simulink model "AFC_FFNN_trainbfg_15_15_15_15_ctr_Nor_July_15"  (R2023a)
settings: Solver=VariableStepAuto  StartTime=0.0  StopTime=10.0  RelTol=1e-3
libraries: neural x66
(part 2 of 3)

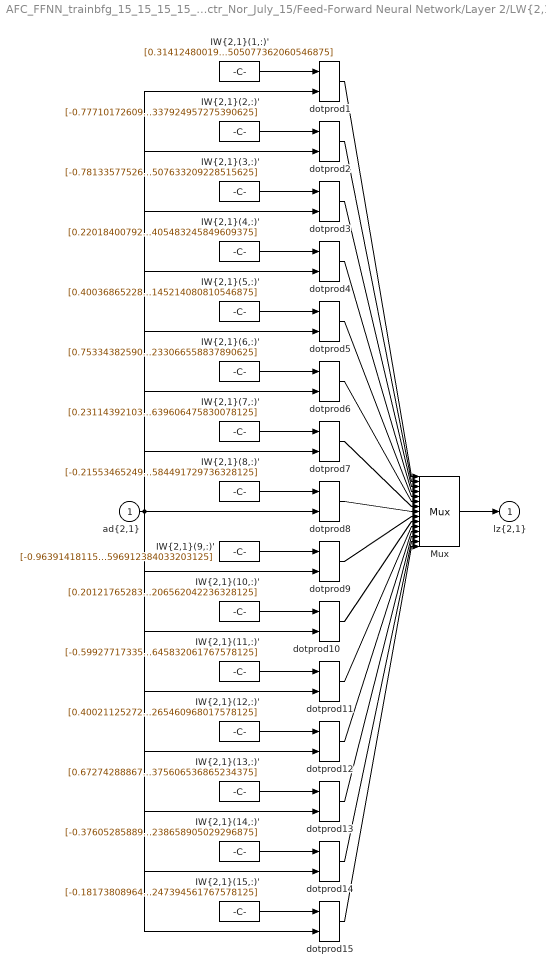
== system AFC_FFNN_trainbfg_15_15_15_15_ctr_Nor_July_15/Feed-Forward Neural Network/Layer 2/LW{2,1} ==
  "ad{2,1}" : Inport  PortDimensions=15
      mask Display: e = 0.06;c1 = [120 230 180]/255;c2 = ([120 230 180]+0)/(256+128);c3 = ([120 230 180]+128)/(256+128);patch([0 1 1 0],[0 0 1 1],c1);patch([0 1 1 1-e 1-e 0+e],[0 0 1 1-e 0+e 0+e],c2);patch([0 0 1 1-e 0+e 0+e],[0 1 1 1-e 1-e 0+e],c3);plot([0 1 1 0 0],[0 0 1 1 0]);
  "IW{2,1}(1,:)'" : Constant  Value=[0.314124800191435848972787425736896693706512451171875;0.761219194780894614638100392767228186130523681640625;-0.171753869070582876332764499238692224025726318359375;0.1327757115322516501265681654331274330615997314453125;0.2459442725020564157745184274972416460514068603515625;0.7167434795542131364953775118920020759105682373046875;-0.4743644560107054264364023765665479004383087158203125;0.9964541018726646992575979311368428170680999755859375;-0.3007178641450372058585571721778251230716705322265625;-0.5061911842499977609577399562112987041473388671875;-0.6212526524824333318264280023868195712566375732421875;-0.32664100949461083445157782989554107189178466796875;-0.164745119790139948889873267035000026226043701171875;-0.37571726232811375467690595542080700397491455078125;-0.9219376696445731322882011227193288505077362060546875]
      mask Display: e = 0.06;c1 = [120 150 230]/255;c2 = ([120 150 230]+0)/383;c3 = ([120 150 230]+128)/383;patch([0 1 1 0],[0 0 1 1],c1);patch([0 1 1 1-e 1-e 0+e],[0 0 1 1-e 0+e 0+e],c2);patch([0 0 1 1-e 0+e 0+e],[0 1 1 1-e 1-e 0+e],c3);plot([0 1 1 0 0],[0 0 1 1 0]);disp('weights');
  "IW{2,1}(10,:)'" : Constant  Value=[0.201217652832927473838253717985935509204864501953125;0.7240782555431468647810788752394728362560272216796875;0.8421596785908558313593630373361520469188690185546875;-1.1825149875412674926877798498026095330715179443359375;-0.31519109748938467507883842699811793863773345947265625;-0.795521501318470658503656522952951490879058837890625;0.0713141598183908431707322961301542818546295166015625;-0.0767485023139631294952778262086212635040283203125;-0.1010553699979890307503183066728524863719940185546875;-0.9567843225283756414256686184671707451343536376953125;-0.7217264190297532078233189167804084718227386474609375;0.50100226468314923433666763230576179921627044677734375;0.87766383555333093990924453464685939252376556396484375;0.29681483600678404410899702270398847758769989013671875;0.2310269064815640149834763406033744104206562042236328125]
      mask Display: e = 0.06;c1 = [120 150 230]/255;c2 = ([120 150 230]+0)/383;c3 = ([120 150 230]+128)/383;patch([0 1 1 0],[0 0 1 1],c1);patch([0 1 1 1-e 1-e 0+e],[0 0 1 1-e 0+e 0+e],c2);patch([0 0 1 1-e 0+e 0+e],[0 1 1 1-e 1-e 0+e],c3);plot([0 1 1 0 0],[0 0 1 1 0]);disp('weights');
  "IW{2,1}(11,:)'" : Constant  Value=[-0.5992771733562098912528881555772386491298675537109375;0.1078487493560353893684577997191809117794036865234375;-0.8945967236389289478637465435895137488842010498046875;-0.0500773407099595058156182858510874211788177490234375;0.8870816241124896972536362227401696145534515380859375;0.74014207030404488563135600998066365718841552734375;-0.6866720030229107596397852830705232918262481689453125;0.2726234239649603097177532617934048175811767578125;0.2078428359638626599092958713299594819545745849609375;0.1188907111891503998180041890009306371212005615234375;-0.469008120701347674952330635278485715389251708984375;-0.37068355488443938128284571575932204723358154296875;-0.123525625729133281538452138192951679229736328125;-0.58507783620791808942840361851267516613006591796875;-0.222821272390497870929948476259596645832061767578125]
      mask Display: e = 0.06;c1 = [120 150 230]/255;c2 = ([120 150 230]+0)/383;c3 = ([120 150 230]+128)/383;patch([0 1 1 0],[0 0 1 1],c1);patch([0 1 1 1-e 1-e 0+e],[0 0 1 1-e 0+e 0+e],c2);patch([0 0 1 1-e 0+e 0+e],[0 1 1 1-e 1-e 0+e],c3);plot([0 1 1 0 0],[0 0 1 1 0]);disp('weights');
  "IW{2,1}(12,:)'" : Constant  Value=[0.4002112527225698546118337617372162640094757080078125;0.6440325108893374395080400063307024538516998291015625;0.2318822635474317994663806530297733843326568603515625;-1.2667374338708261571895263841724954545497894287109375;-0.5533384432674870456736471169278956949710845947265625;-0.26613616681114093953652854906977154314517974853515625;0.3727253587085710417881045941612683236598968505859375;0.48813811599891376857840441516600549221038818359375;0.6001589125458657303369136570836417376995086669921875;-0.0802101438462316795874329500293242745101451873779296875;0.65367435221139091883202354438253678381443023681640625;-1.0458216791451082627872892771847546100616455078125;-1.3193113394946169858457096779602579772472381591796875;-0.330369571278571971806314877539989538490772247314453125;0.997369857636166035064206880633719265460968017578125]
      mask Display: e = 0.06;c1 = [120 150 230]/255;c2 = ([120 150 230]+0)/383;c3 = ([120 150 230]+128)/383;patch([0 1 1 0],[0 0 1 1],c1);patch([0 1 1 1-e 1-e 0+e],[0 0 1 1-e 0+e 0+e],c2);patch([0 0 1 1-e 0+e 0+e],[0 1 1 1-e 1-e 0+e],c3);plot([0 1 1 0 0],[0 0 1 1 0]);disp('weights');
  "IW{2,1}(13,:)'" : Constant  Value=[0.67274288867184051099457064992748200893402099609375;0.189393636354295846757622712175361812114715576171875;-0.510549226010743151249471338815055787563323974609375;1.104023685506638319253625013516284525394439697265625;0.8308657357789719366536473899031989276409149169921875;0.367241219801807627920453569458913989365100860595703125;0.8655885705956922748782744747586548328399658203125;-0.0858121130468900705778878545970655977725982666015625;-0.8378375318602981902671444913721643388271331787109375;-0.88685905025613409602414094479172490537166595458984375;0.275859743807580104490995154264965094625949859619140625;0.2062969216335570621367878629826009273529052734375;1.1086902941997625049452835810370743274688720703125;0.442383535765201452161221595815732143819332122802734375;0.95884080775527402717983704860671423375606536865234375]
      mask Display: e = 0.06;c1 = [120 150 230]/255;c2 = ([120 150 230]+0)/383;c3 = ([120 150 230]+128)/383;patch([0 1 1 0],[0 0 1 1],c1);patch([0 1 1 1-e 1-e 0+e],[0 0 1 1-e 0+e 0+e],c2);patch([0 0 1 1-e 0+e 0+e],[0 1 1 1-e 1-e 0+e],c3);plot([0 1 1 0 0],[0 0 1 1 0]);disp('weights');
  "IW{2,1}(14,:)'" : Constant  Value=[-0.3760528588983949038748733073589392006397247314453125;-0.3766582837641696546171488080290146172046661376953125;0.9248846167847240007375830828095786273479461669921875;-0.8676145111114246244454761836095713078975677490234375;0.157385168877649583851763281927560456097126007080078125;-0.4984382819952763998827549585257656872272491455078125;-0.07612045846803727755514046293683350086212158203125;0.1706855767497774678531641256995499134063720703125;0.6769974800018092597753138761618174612522125244140625;0.5403602376259268869063134843599982559680938720703125;-2.3605068409971039500305778346955776214599609375;-0.16106471547288514489792987660621292889118194580078125;-0.369042109842184939960674228132120333611965179443359375;-0.95704290874445641090773051473661325871944427490234375;0.843577088247318140901143124210648238658905029296875]
      mask Display: e = 0.06;c1 = [120 150 230]/255;c2 = ([120 150 230]+0)/383;c3 = ([120 150 230]+128)/383;patch([0 1 1 0],[0 0 1 1],c1);patch([0 1 1 1-e 1-e 0+e],[0 0 1 1-e 0+e 0+e],c2);patch([0 0 1 1-e 0+e 0+e],[0 1 1 1-e 1-e 0+e],c3);plot([0 1 1 0 0],[0 0 1 1 0]);disp('weights');
  "IW{2,1}(15,:)'" : Constant  Value=[-0.1817380896437239545804231966030783951282501220703125;-0.819076525749918626928547382703982293605804443359375;-0.703422130964734382274627932929433882236480712890625;-0.94939269002778214900928333008778281509876251220703125;-0.896269677871021741566437412984669208526611328125;-0.3356003910290790148707174012088216841220855712890625;-0.2214840900786894106744284727028571069240570068359375;-0.4191414392946388733918183788773603737354278564453125;-0.2687179919619584467227468849159777164459228515625;0.98276969821900905799338943324983119964599609375;-0.0363505221006390488724946408183313906192779541015625;-0.55328677456039410120780530633055604994297027587890625;0.89155338038898801489295919964206404983997344970703125;-0.11752903231500504144246832538556191138923168182373046875;-0.79833567739331734447461030867998488247394561767578125]
      mask Display: e = 0.06;c1 = [120 150 230]/255;c2 = ([120 150 230]+0)/383;c3 = ([120 150 230]+128)/383;patch([0 1 1 0],[0 0 1 1],c1);patch([0 1 1 1-e 1-e 0+e],[0 0 1 1-e 0+e 0+e],c2);patch([0 0 1 1-e 0+e 0+e],[0 1 1 1-e 1-e 0+e],c3);plot([0 1 1 0 0],[0 0 1 1 0]);disp('weights');
  "IW{2,1}(2,:)'" : Constant  Value=[-0.7771017260971981865935731548233889043331146240234375;-0.989689411673975616423604151350446045398712158203125;0.85939642766992552225246981834061443805694580078125;-0.61030381879570694270142894310993142426013946533203125;0.30497898667072576017744722776114940643310546875;0.092222522227818071183236270371708087623119354248046875;-0.005466530920209766719608523999340832233428955078125;0.8236928328595840564929631000268273055553436279296875;0.0456944657569839929323052274412475526332855224609375;0.8261448944639935287881371550611220300197601318359375;0.429014213658457210787133817575522698462009429931640625;-0.32131717688586680647944149313843809068202972412109375;-0.52240941017245867694640537592931650578975677490234375;0.29152713968148391554535692193894647061824798583984375;0.494308555574343666538794650477939285337924957275390625]
      mask Display: e = 0.06;c1 = [120 150 230]/255;c2 = ([120 150 230]+0)/383;c3 = ([120 150 230]+128)/383;patch([0 1 1 0],[0 0 1 1],c1);patch([0 1 1 1-e 1-e 0+e],[0 0 1 1-e 0+e 0+e],c2);patch([0 0 1 1-e 0+e 0+e],[0 1 1 1-e 1-e 0+e],c3);plot([0 1 1 0 0],[0 0 1 1 0]);disp('weights');
  "IW{2,1}(3,:)'" : Constant  Value=[-0.7813357752653991017410817221389152109622955322265625;0.2884373573340142105081440604408271610736846923828125;-0.1790504980917517752203593772719614207744598388671875;-0.62459444844897393789295847454923205077648162841796875;0.9792166972620892639866951867588795721530914306640625;-0.05772109104215349117961153524447581730782985687255859375;-0.0859133263877100983307855130988173186779022216796875;-0.903421362694661223002867700415663421154022216796875;-0.3519069100123857207762512189219705760478973388671875;0.68567142254128310430161263866466470062732696533203125;0.427114206938296436799618049917626194655895233154296875;-0.1887415273689747596819188402150757610797882080078125;0.08611314277500585478986039333904045633971691131591796875;0.9918392466822412156801647142856381833553314208984375;-0.8345158850484593049401382813812233507633209228515625]
      mask Display: e = 0.06;c1 = [120 150 230]/255;c2 = ([120 150 230]+0)/383;c3 = ([120 150 230]+128)/383;patch([0 1 1 0],[0 0 1 1],c1);patch([0 1 1 1-e 1-e 0+e],[0 0 1 1-e 0+e 0+e],c2);patch([0 0 1 1-e 0+e 0+e],[0 1 1 1-e 1-e 0+e],c3);plot([0 1 1 0 0],[0 0 1 1 0]);disp('weights');
  "IW{2,1}(4,:)'" : Constant  Value=[0.22018400792110437436122083454392850399017333984375;0.6991144072415418353472205126308836042881011962890625;0.3099402980647762984034443434211425483226776123046875;0.061498952364746749255086655239210813306272029876708984375;0.439963017584670768034271759461262263357639312744140625;0.53700087765160320341095712137757800519466400146484375;-0.9259617635520160927597999034333042800426483154296875;0.6153389276731864310221453706617467105388641357421875;-0.4045481598141231760479286094778217375278472900390625;0.70229649611518774054985669863526709377765655517578125;-1.0632415478873624703481937103788368403911590576171875;1.037732974579840483642101389705203473567962646484375;-0.56732075540575477301530327167711220681667327880859375;0.03649661653649223513884436442822334356606006622314453125;0.6470024656570847465530960107571445405483245849609375]
      mask Display: e = 0.06;c1 = [120 150 230]/255;c2 = ([120 150 230]+0)/383;c3 = ([120 150 230]+128)/383;patch([0 1 1 0],[0 0 1 1],c1);patch([0 1 1 1-e 1-e 0+e],[0 0 1 1-e 0+e 0+e],c2);patch([0 0 1 1-e 0+e 0+e],[0 1 1 1-e 1-e 0+e],c3);plot([0 1 1 0 0],[0 0 1 1 0]);disp('weights');
  "IW{2,1}(5,:)'" : Constant  Value=[0.4003686522850926632344226163695566356182098388671875;0.7154922757569484037531992726144380867481231689453125;-0.55451457198497333678233189857564866542816162109375;-0.701016426748160892401529054041020572185516357421875;0.2719693029116949656298629633965902030467987060546875;0.3452701580345747256473032393842004239559173583984375;-0.9904793588654232650014819228090345859527587890625;0.421753225196830339172038293327204883098602294921875;-0.6134849306530993917618843624950386583805084228515625;0.6205332793438713689937458184431307017803192138671875;-0.2900360464848421582217952163773588836193084716796875;-0.8601594396824143728963463217951357364654541015625;-0.7387104842103118240714820785797201097011566162109375;-0.64540323855050463208726796437986195087432861328125;-0.2133330335187888504577813364448957145214080810546875]
      mask Display: e = 0.06;c1 = [120 150 230]/255;c2 = ([120 150 230]+0)/383;c3 = ([120 150 230]+128)/383;patch([0 1 1 0],[0 0 1 1],c1);patch([0 1 1 1-e 1-e 0+e],[0 0 1 1-e 0+e 0+e],c2);patch([0 0 1 1-e 0+e 0+e],[0 1 1 1-e 1-e 0+e],c3);plot([0 1 1 0 0],[0 0 1 1 0]);disp('weights');
  "IW{2,1}(6,:)'" : Constant  Value=[0.7533438259077460674717485744622536003589630126953125;-0.1622850437559437697387920707114972174167633056640625;-0.2221844078714447778821750034694559872150421142578125;0.54429151285718668784596729892655275762081146240234375;1.00787934291988801049910762230865657329559326171875;0.3163128591791328769744495730265043675899505615234375;0.2893143771285426879558144719339907169342041015625;0.9802256885177147438525935285724699497222900390625;-0.3613982857657287439678839291445910930633544921875;-0.90323576071038391699374869858729653060436248779296875;1.52266978362477178876588368439115583896636962890625;0.414545013788929994635878983899601735174655914306640625;-0.25805726547611007593019394334987737238407135009765625;0.79414819953845261490954499095096252858638763427734375;0.465672824324343537227832712233066558837890625]
      mask Display: e = 0.06;c1 = [120 150 230]/255;c2 = ([120 150 230]+0)/383;c3 = ([120 150 230]+128)/383;patch([0 1 1 0],[0 0 1 1],c1);patch([0 1 1 1-e 1-e 0+e],[0 0 1 1-e 0+e 0+e],c2);patch([0 0 1 1-e 0+e 0+e],[0 1 1 1-e 1-e 0+e],c3);plot([0 1 1 0 0],[0 0 1 1 0]);disp('weights');
  "IW{2,1}(7,:)'" : Constant  Value=[0.23114392103916969745114329271018505096435546875;0.9635763073263967637416271827532909810543060302734375;-0.1671208207308916282585187218501232564449310302734375;0.06329895739177394953234312424683594144880771636962890625;-0.378452929134685034373575263089151121675968170166015625;0.11958422424242327875010261095667374320328235626220703125;-0.607419333399665362094310694374144077301025390625;0.0111096917961808205888019074336625635623931884765625;-0.8105754243397400582438194760470651090145111083984375;0.318929817605345056197307940237806178629398345947265625;-0.7900852178016195548337918808101676404476165771484375;-0.21373528018232745839810604593367315828800201416015625;-0.5969408965863836069587478050380013883113861083984375;-0.90852813610887828144058175894315354526042938232421875;-0.287242937260107134012088181407307274639606475830078125]
      mask Display: e = 0.06;c1 = [120 150 230]/255;c2 = ([120 150 230]+0)/383;c3 = ([120 150 230]+128)/383;patch([0 1 1 0],[0 0 1 1],c1);patch([0 1 1 1-e 1-e 0+e],[0 0 1 1-e 0+e 0+e],c2);patch([0 0 1 1-e 0+e 0+e],[0 1 1 1-e 1-e 0+e],c3);plot([0 1 1 0 0],[0 0 1 1 0]);disp('weights');
  "IW{2,1}(8,:)'" : Constant  Value=[-0.2155346524932839624710823045461438596248626708984375;0.890530830596826472600469060125760734081268310546875;-0.9467920414380841531709620539913885295391082763671875;-0.434011281189908115774045427315286360681056976318359375;0.26579035938519302018079315530485473573207855224609375;0.2172980620921392269639937921965611167252063751220703125;0.292716250101574093633871598285622894763946533203125;0.1305612562825471112404329687706194818019866943359375;-0.871055828832263845384886735701002180576324462890625;-0.17721316472024450927591487925383262336254119873046875;-0.71934773715706235019951009235228411853313446044921875;0.25931984951627884417035829756059683859348297119140625;0.21468822963550027171919509783037938177585601806640625;0.16340570924226149873703661796753294765949249267578125;-0.81406715037500021470151523317326791584491729736328125]
      mask Display: e = 0.06;c1 = [120 150 230]/255;c2 = ([120 150 230]+0)/383;c3 = ([120 150 230]+128)/383;patch([0 1 1 0],[0 0 1 1],c1);patch([0 1 1 1-e 1-e 0+e],[0 0 1 1-e 0+e 0+e],c2);patch([0 0 1 1-e 0+e 0+e],[0 1 1 1-e 1-e 0+e],c3);plot([0 1 1 0 0],[0 0 1 1 0]);disp('weights');
  "IW{2,1}(9,:)'" : Constant  Value=[-0.96391418115658300536097158328630030155181884765625;0.510168063185229225808825503918342292308807373046875;0.312107034951037309866705982130952179431915283203125;0.33415533498262950384827263405895791947841644287109375;0.159088574682244077163062456747866235673427581787109375;0.303936777339137431663829147510114125907421112060546875;-0.06134999454679768149389929021708667278289794921875;-0.769981108969951311138402161304838955402374267578125;-0.5287401885702369686015344996121712028980255126953125;-0.0309998749507064234876008157471005688421428203582763671875;0.18321056239390876019257348161772824823856353759765625;0.0783758268001817637316008813286316581070423126220703125;0.1645435635146068609202529842150397598743438720703125;-1.1439631090601272145335087770945392549037933349609375;0.74931802165753680355919641442596912384033203125]
      mask Display: e = 0.06;c1 = [120 150 230]/255;c2 = ([120 150 230]+0)/383;c3 = ([120 150 230]+128)/383;patch([0 1 1 0],[0 0 1 1],c1);patch([0 1 1 1-e 1-e 0+e],[0 0 1 1-e 0+e 0+e],c2);patch([0 0 1 1-e 0+e 0+e],[0 1 1 1-e 1-e 0+e],c3);plot([0 1 1 0 0],[0 0 1 1 0]);disp('weights');
  Mux : Mux  Inputs=15
      mask Display: e = 0.06;c1 = [120 150 230]/255;c2 = ([120 150 230]+0)/383;c3 = ([120 150 230]+128)/383;patch([0 1 1 0],[0 0 1 1],c1);patch([0 1 1 1-e 1-e 0+e],[0 0 1 1-e 0+e 0+e],c2);patch([0 0 1 1-e 0+e 0+e],[0 1 1 1-e 1-e 0+e],c3);plot([0 1 1 0 0],[0 0 1 1 0]);disp('Mux');
  dotprod{1..15} (15 alike) : neural/Weight Functions/dotprod
  "lz{2,1}" : Outport
      mask Display: e = 0.06;c1 = [120 230 180]/255;c2 = ([120 230 180]+0)/(256+128);c3 = ([120 230 180]+128)/(256+128);patch([0 1 1 0],[0 0 1 1],c1);patch([0 1 1 1-e 1-e 0+e],[0 0 1 1-e 0+e 0+e],c2);patch([0 0 1 1-e 0+e 0+e],[0 1 1 1-e 1-e 0+e],c3);plot([0 1 1 0 0],[0 0 1 1 0]);
  wires:
  "IW{2,1}(1,:)'"/1 -> dotprod1/1
  "ad{2,1}"/1 -> dotprod1/2, dotprod2/2, dotprod3/2, dotprod4/2, dotprod5/2, dotprod6/2, dotprod7/2, dotprod8/2, dotprod9/2, dotprod10/2, dotprod11/2, dotprod12/2, dotprod13/2, dotprod14/2, dotprod15/2
  dotprod1/1 -> Mux/1
  "IW{2,1}(2,:)'"/1 -> dotprod2/1
  dotprod2/1 -> Mux/2
  "IW{2,1}(3,:)'"/1 -> dotprod3/1
  dotprod3/1 -> Mux/3
  "IW{2,1}(4,:)'"/1 -> dotprod4/1
  dotprod4/1 -> Mux/4
  "IW{2,1}(5,:)'"/1 -> dotprod5/1
  dotprod5/1 -> Mux/5
  "IW{2,1}(6,:)'"/1 -> dotprod6/1
  dotprod6/1 -> Mux/6
  "IW{2,1}(7,:)'"/1 -> dotprod7/1
  dotprod7/1 -> Mux/7
  "IW{2,1}(8,:)'"/1 -> dotprod8/1
  dotprod8/1 -> Mux/8
  "IW{2,1}(9,:)'"/1 -> dotprod9/1
  dotprod9/1 -> Mux/9
  "IW{2,1}(10,:)'"/1 -> dotprod10/1
  dotprod10/1 -> Mux/10
  "IW{2,1}(11,:)'"/1 -> dotprod11/1
  dotprod11/1 -> Mux/11
  "IW{2,1}(12,:)'"/1 -> dotprod12/1
  dotprod12/1 -> Mux/12
  "IW{2,1}(13,:)'"/1 -> dotprod13/1
  dotprod13/1 -> Mux/13
  "IW{2,1}(14,:)'"/1 -> dotprod14/1
  dotprod14/1 -> Mux/14
  "IW{2,1}(15,:)'"/1 -> dotprod15/1
  dotprod15/1 -> Mux/15
  Mux/1 -> "lz{2,1}"/1

== system AFC_FFNN_trainbfg_15_15_15_15_ctr_Nor_July_15/Feed-Forward Neural Network/Layer 3/Delays 1 ==
  "p{3}" : Inport  PortDimensions=15
      mask Display: e = 0.06;c1 = [120 230 180]/255;c2 = ([120 230 180]+0)/(256+128);c3 = ([120 230 180]+128)/(256+128);patch([0 1 1 0],[0 0 1 1],c1);patch([0 1 1 1-e 1-e 0+e],[0 0 1 1-e 0+e 0+e],c2);patch([0 0 1 1-e 0+e 0+e],[0 1 1 1-e 1-e 0+e],c3);plot([0 1 1 0 0],[0 0 1 1 0]);
  mux : Mux  Inputs=1
      mask Display: e = 0.06;c1 = [120 150 230]/255;c2 = ([120 150 230]+0)/383;c3 = ([120 150 230]+128)/383;patch([0 1 1 0],[0 0 1 1],c1);patch([0 1 1 1-e 1-e 0+e],[0 0 1 1-e 0+e 0+e],c2);patch([0 0 1 1-e 0+e 0+e],[0 1 1 1-e 1-e 0+e],c3);plot([0 1 1 0 0],[0 0 1 1 0]);disp('Mux')
  "pd{3,2}" : Outport
      mask Display: e = 0.06;c1 = [120 230 180]/255;c2 = ([120 230 180]+0)/(256+128);c3 = ([120 230 180]+128)/(256+128);patch([0 1 1 0],[0 0 1 1],c1);patch([0 1 1 1-e 1-e 0+e],[0 0 1 1-e 0+e 0+e],c2);patch([0 0 1 1-e 0+e 0+e],[0 1 1 1-e 1-e 0+e],c3);plot([0 1 1 0 0],[0 0 1 1 0]);
  wires:
  "p{3}"/1 -> mux/1
  mux/1 -> "pd{3,2}"/1

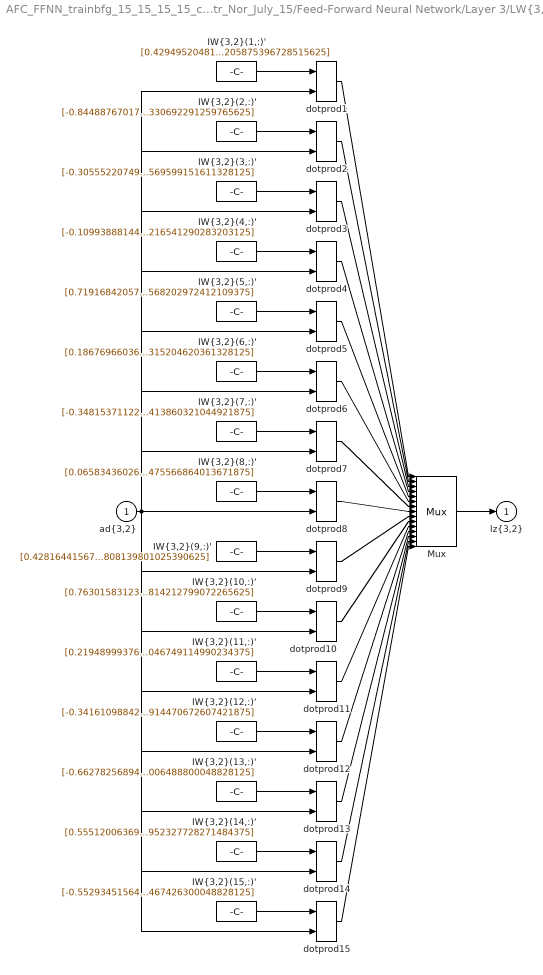
== system AFC_FFNN_trainbfg_15_15_15_15_ctr_Nor_July_15/Feed-Forward Neural Network/Layer 3/LW{3,2} ==
  "ad{3,2}" : Inport  PortDimensions=15
      mask Display: e = 0.06;c1 = [120 230 180]/255;c2 = ([120 230 180]+0)/(256+128);c3 = ([120 230 180]+128)/(256+128);patch([0 1 1 0],[0 0 1 1],c1);patch([0 1 1 1-e 1-e 0+e],[0 0 1 1-e 0+e 0+e],c2);patch([0 0 1 1-e 0+e 0+e],[0 1 1 1-e 1-e 0+e],c3);plot([0 1 1 0 0],[0 0 1 1 0]);
  "IW{3,2}(1,:)'" : Constant  Value=[0.4294952048164033531207905980409123003482818603515625;-0.612678315643889082053874517441727221012115478515625;-0.41663875275807360498703246776130981743335723876953125;-0.5383112997877292915660518701770342886447906494140625;-0.493758505920776968878271873109042644500732421875;-0.4693349103558774881861381800263188779354095458984375;0.2066025308635509871724167396678240038454532623291015625;0.465960500926316967262863499854574911296367645263671875;0.7996983840137072974130205693654716014862060546875;-0.01536163101939420905228672609155182726681232452392578125;-0.4735079014873659897233437732211314141750335693359375;0.048185810994904536286309593151599983684718608856201171875;0.6244275337507332324094022624194622039794921875;-0.11131049593420443144520248779372195713222026824951171875;0.63703528847606760709965101341367699205875396728515625]
      mask Display: e = 0.06;c1 = [120 150 230]/255;c2 = ([120 150 230]+0)/383;c3 = ([120 150 230]+128)/383;patch([0 1 1 0],[0 0 1 1],c1);patch([0 1 1 1-e 1-e 0+e],[0 0 1 1-e 0+e 0+e],c2);patch([0 0 1 1-e 0+e 0+e],[0 1 1 1-e 1-e 0+e],c3);plot([0 1 1 0 0],[0 0 1 1 0]);disp('weights');
  "IW{3,2}(10,:)'" : Constant  Value=[0.7630158312346824178717952236183919012546539306640625;0.1984316808513547913950247902903356589376926422119140625;-0.82423007976842577182452487249975092709064483642578125;1.0226211205456607888919506876845844089984893798828125;0.739625288102554900859786357614211738109588623046875;-0.2417860871958233681677796766962273977696895599365234375;0.44995290604095483644186970195733010768890380859375;0.9976633534078038767489715610281564295291900634765625;0.26713856145543279918541657025343738496303558349609375;-0.32276591319424319248554411387885920703411102294921875;-0.0162040947031620863327816550736315548419952392578125;0.917692798491053896015046120737679302692413330078125;-0.89634757541265097646743242876254953444004058837890625;-0.07517365498519591737736078584930510260164737701416015625;0.635019639107901046060078442678786814212799072265625]
      mask Display: e = 0.06;c1 = [120 150 230]/255;c2 = ([120 150 230]+0)/383;c3 = ([120 150 230]+128)/383;patch([0 1 1 0],[0 0 1 1],c1);patch([0 1 1 1-e 1-e 0+e],[0 0 1 1-e 0+e 0+e],c2);patch([0 0 1 1-e 0+e 0+e],[0 1 1 1-e 1-e 0+e],c3);plot([0 1 1 0 0],[0 0 1 1 0]);disp('weights');
  "IW{3,2}(11,:)'" : Constant  Value=[0.219489993767322477680181691539473831653594970703125;-0.052080718123408677178165504528806195594370365142822265625;0.8628210117321575278737100234138779342174530029296875;-0.35442212669388017953764347112155519425868988037109375;-0.1590347864723649085050283247255720198154449462890625;1.363795369435750526321271536289714276790618896484375;-0.001054289977101671195447440965153873548842966556549072265625;0.36148378499434208332985463130171410739421844482421875;0.0823384967626836772325304991682060062885284423828125;-0.238644865874834188890218911183183081448078155517578125;0.0105659440395431403203474474139511585235595703125;-0.61124435721228354001510751913883723318576812744140625;1.2260791554399050884427424534806050360202789306640625;-0.27460477604993294153956640002434141933917999267578125;-0.1981978971777476894455816136542125605046749114990234375]
      mask Display: e = 0.06;c1 = [120 150 230]/255;c2 = ([120 150 230]+0)/383;c3 = ([120 150 230]+128)/383;patch([0 1 1 0],[0 0 1 1],c1);patch([0 1 1 1-e 1-e 0+e],[0 0 1 1-e 0+e 0+e],c2);patch([0 0 1 1-e 0+e 0+e],[0 1 1 1-e 1-e 0+e],c3);plot([0 1 1 0 0],[0 0 1 1 0]);disp('weights');
  "IW{3,2}(12,:)'" : Constant  Value=[-0.341610988428120432303103370941244065761566162109375;-0.00116667452464628662416046278593739771167747676372528076171875;0.20784158680182518441625916238990612328052520751953125;-0.07459817549295848226886818110870081000030040740966796875;0.629697204521345810235288809053599834442138671875;0.8865714109056013203513657572329975664615631103515625;-0.321810848017774986384864632782409898936748504638671875;0.432273916709559336002399732024059630930423736572265625;0.379607625872108778164459863546653650701045989990234375;0.57171490814849323935931124651688151061534881591796875;0.1472744754105674847011187011958099901676177978515625;0.460402115286616286926602015228127129375934600830078125;0.10741000111703445651922805836875340901315212249755859375;-0.9041271141678794975860000704415142536163330078125;-0.443306183838275635888948045248980633914470672607421875]
      mask Display: e = 0.06;c1 = [120 150 230]/255;c2 = ([120 150 230]+0)/383;c3 = ([120 150 230]+128)/383;patch([0 1 1 0],[0 0 1 1],c1);patch([0 1 1 1-e 1-e 0+e],[0 0 1 1-e 0+e 0+e],c2);patch([0 0 1 1-e 0+e 0+e],[0 1 1 1-e 1-e 0+e],c3);plot([0 1 1 0 0],[0 0 1 1 0]);disp('weights');
  "IW{3,2}(13,:)'" : Constant  Value=[-0.66278256894771292451196131878532469272613525390625;-1.672291331705338279789430089294910430908203125;-0.38098498454672913293705960313673131167888641357421875;0.2983177358270283630048425038694404065608978271484375;-0.9202199705157365627883336856029927730560302734375;-1.6388389412374377851477902368060313165187835693359375;-0.7448345748382845243895644671283662319183349609375;0.77021932698641226711089302625623531639575958251953125;-1.2315395326944422738080220369738526642322540283203125;0.1128863476450611968981974087000708095729351043701171875;-0.8513836971448534018946929791127331554889678955078125;-1.0258859877296082618869377256487496197223663330078125;-1.39387245449321373058637618669308722019195556640625;-0.8687091691382116120934142600162886083126068115234375;-0.7700777924421189357673256381531246006488800048828125]
      mask Display: e = 0.06;c1 = [120 150 230]/255;c2 = ([120 150 230]+0)/383;c3 = ([120 150 230]+128)/383;patch([0 1 1 0],[0 0 1 1],c1);patch([0 1 1 1-e 1-e 0+e],[0 0 1 1-e 0+e 0+e],c2);patch([0 0 1 1-e 0+e 0+e],[0 1 1 1-e 1-e 0+e],c3);plot([0 1 1 0 0],[0 0 1 1 0]);disp('weights');
  "IW{3,2}(14,:)'" : Constant  Value=[0.555120063696358467808522618724964559078216552734375;-0.09894607580444551853116053052872302941977977752685546875;0.305756013218437872058785842455108650028705596923828125;-0.2069757069841939578491718521036091260612010955810546875;0.5236794338292234396448066036100499331951141357421875;0.781578562966814160972717218101024627685546875;0.925770941019874893385122049949131906032562255859375;-0.226360645757738065952935357927344739437103271484375;-0.62344387744347640190056836217991076409816741943359375;-0.54223723805426360389247975035686977207660675048828125;-0.3542426822873754321818751122918911278247833251953125;-0.10062609396851908416525844813804724253714084625244140625;-0.60891512989643270525874640952679328620433807373046875;-0.053775078503994037937285810357934678904712200164794921875;-0.7076681573893226495641783913015387952327728271484375]
      mask Display: e = 0.06;c1 = [120 150 230]/255;c2 = ([120 150 230]+0)/383;c3 = ([120 150 230]+128)/383;patch([0 1 1 0],[0 0 1 1],c1);patch([0 1 1 1-e 1-e 0+e],[0 0 1 1-e 0+e 0+e],c2);patch([0 0 1 1-e 0+e 0+e],[0 1 1 1-e 1-e 0+e],c3);plot([0 1 1 0 0],[0 0 1 1 0]);disp('weights');
  "IW{3,2}(15,:)'" : Constant  Value=[-0.552934515642912405297693112515844404697418212890625;-0.30075123633298284087089768945588730275630950927734375;-0.08501069722579314424937280136873596347868442535400390625;0.72562881316305161139013080173754133284091949462890625;-0.079368032880180461319241658202372491359710693359375;-0.7423600633093923040206618679803796112537384033203125;0.408580117977064116718821651375037617981433868408203125;-0.6116357762143371790131141096935607492923736572265625;0.08264039362662288501493179637691355310380458831787109375;0.347506445741584124586864845696254633367061614990234375;-0.9886562132901974830900826418655924499034881591796875;0.94918588506836709672853658048552460968494415283203125;1.0474680392741293477598674144246615469455718994140625;0.53384758038892687892484900658018887042999267578125;-0.2372585876275876970442624269708176143467426300048828125]
      mask Display: e = 0.06;c1 = [120 150 230]/255;c2 = ([120 150 230]+0)/383;c3 = ([120 150 230]+128)/383;patch([0 1 1 0],[0 0 1 1],c1);patch([0 1 1 1-e 1-e 0+e],[0 0 1 1-e 0+e 0+e],c2);patch([0 0 1 1-e 0+e 0+e],[0 1 1 1-e 1-e 0+e],c3);plot([0 1 1 0 0],[0 0 1 1 0]);disp('weights');
  "IW{3,2}(2,:)'" : Constant  Value=[-0.8448876701768590624652688347850926220417022705078125;-0.0538388952155621769435356327448971569538116455078125;-0.2690932818904168133400389706366695463657379150390625;-0.98017730775724920544433871327782981097698211669921875;-0.37904000714715646580543761956505477428436279296875;-0.31094857201915060418428993216366507112979888916015625;0.219769365539062899728151023737154901027679443359375;-0.5910279837821719173263090851833112537860870361328125;-0.6862175631530516017875243051094003021717071533203125;-0.6523710301420024837426581143517978489398956298828125;-0.34206029681594340985384405939839780330657958984375;0.239587834758158368941849403199739754199981689453125;0.6623164964936882892487801655079238116741180419921875;0.6427690120268698681371688508079387247562408447265625;-0.81383550246944358352862991523579694330692291259765625]
      mask Display: e = 0.06;c1 = [120 150 230]/255;c2 = ([120 150 230]+0)/383;c3 = ([120 150 230]+128)/383;patch([0 1 1 0],[0 0 1 1],c1);patch([0 1 1 1-e 1-e 0+e],[0 0 1 1-e 0+e 0+e],c2);patch([0 0 1 1-e 0+e 0+e],[0 1 1 1-e 1-e 0+e],c3);plot([0 1 1 0 0],[0 0 1 1 0]);disp('weights');
  "IW{3,2}(3,:)'" : Constant  Value=[-0.3055522074982641722584730814560316503047943115234375;0.5665869649025629950500615450437180697917938232421875;0.071199336634411081181639247006387449800968170166015625;0.288339577238945654613644364872016012668609619140625;0.4106526758379249741892635938711464405059814453125;0.385876628268256360865251508585060946643352508544921875;0.0914900373172624625794924213550984859466552734375;-0.36248110666585464656463955179788172245025634765625;0.09184886789510234017530621031255577690899372100830078125;0.0193957862645101654364143684006194234825670719146728515625;0.7238374758794805519102055768598802387714385986328125;0.3132733782825980473063509634812362492084503173828125;-0.83750985046541781553486316624912433326244354248046875;0.604369831840676940970524810836650431156158447265625;0.80651036891984262400256966429878957569599151611328125]
      mask Display: e = 0.06;c1 = [120 150 230]/255;c2 = ([120 150 230]+0)/383;c3 = ([120 150 230]+128)/383;patch([0 1 1 0],[0 0 1 1],c1);patch([0 1 1 1-e 1-e 0+e],[0 0 1 1-e 0+e 0+e],c2);patch([0 0 1 1-e 0+e 0+e],[0 1 1 1-e 1-e 0+e],c3);plot([0 1 1 0 0],[0 0 1 1 0]);disp('weights');
  "IW{3,2}(4,:)'" : Constant  Value=[-0.1099388814495494415268694865517318248748779296875;0.6187779335822465309746576167526654899120330810546875;0.516841841257460021807901284773834049701690673828125;-0.524964717876703179655351050314493477344512939453125;-0.362800002813841171445119471172802150249481201171875;-0.8831515396491536051826187758706510066986083984375;-0.4767342557674947300938583794049918651580810546875;0.2933585055759546644793545056018047034740447998046875;0.0045669865725361802333281957544386386871337890625;-0.0906953734773459085971580861951224505901336669921875;0.706787173330524876035951820085756480693817138671875;-0.5622356034924251844131504185497760772705078125;0.348462004036084405100837102509103715419769287109375;-0.0357165571439550522114814157248474657535552978515625;-0.1130256756824661312776925115031190216541290283203125]
      mask Display: e = 0.06;c1 = [120 150 230]/255;c2 = ([120 150 230]+0)/383;c3 = ([120 150 230]+128)/383;patch([0 1 1 0],[0 0 1 1],c1);patch([0 1 1 1-e 1-e 0+e],[0 0 1 1-e 0+e 0+e],c2);patch([0 0 1 1-e 0+e 0+e],[0 1 1 1-e 1-e 0+e],c3);plot([0 1 1 0 0],[0 0 1 1 0]);disp('weights');
  "IW{3,2}(5,:)'" : Constant  Value=[0.719168420574110456300331861712038516998291015625;0.0847737795487171208463905713870190083980560302734375;-0.141553298693671780750236166568356566131114959716796875;0.6788606635025420388274142169393599033355712890625;0.8932262043684249253061580020585097372531890869140625;-0.241966142969885555924491882251459173858165740966796875;-0.739255956912197031982714179321192204952239990234375;-0.7400967432848950533497145443107001483440399169921875;-0.2422206485527137742597147962442249990999698638916015625;0.5005674876542745010965518304146826267242431640625;-0.9594575603270742991668385002412833273410797119140625;0.197719552715467539183435974337044171988964080810546875;0.3366654479273407662986983268638141453266143798828125;-0.13031606394009942473388719008653424680233001708984375;0.73395107780940482822273907004273496568202972412109375]
      mask Display: e = 0.06;c1 = [120 150 230]/255;c2 = ([120 150 230]+0)/383;c3 = ([120 150 230]+128)/383;patch([0 1 1 0],[0 0 1 1],c1);patch([0 1 1 1-e 1-e 0+e],[0 0 1 1-e 0+e 0+e],c2);patch([0 0 1 1-e 0+e 0+e],[0 1 1 1-e 1-e 0+e],c3);plot([0 1 1 0 0],[0 0 1 1 0]);disp('weights');
  "IW{3,2}(6,:)'" : Constant  Value=[0.186769660362741785064599753241054713726043701171875;0.5620259810922336729532844401546753942966461181640625;-0.11959347594884039978069267817772924900054931640625;0.2975256040824234560204786248505115509033203125;-0.47897995742988808132167832809500396251678466796875;-0.1724617171978507224050503054968430660665035247802734375;-0.312929225364951768550980659711058251559734344482421875;0.71983954572869823795855381831643171608448028564453125;0.4738927604266383042386223678477108478546142578125;0.59121953726546350171844323995173908770084381103515625;-0.132711710780250680130620821728371083736419677734375;0.88317009485144382097132620401680469512939453125;-0.390049186299380734599395736950100399553775787353515625;0.2089508793613176484971205582041875459253787994384765625;-0.7894884252939420310468676689197309315204620361328125]
      mask Display: e = 0.06;c1 = [120 150 230]/255;c2 = ([120 150 230]+0)/383;c3 = ([120 150 230]+128)/383;patch([0 1 1 0],[0 0 1 1],c1);patch([0 1 1 1-e 1-e 0+e],[0 0 1 1-e 0+e 0+e],c2);patch([0 0 1 1-e 0+e 0+e],[0 1 1 1-e 1-e 0+e],c3);plot([0 1 1 0 0],[0 0 1 1 0]);disp('weights');
  "IW{3,2}(7,:)'" : Constant  Value=[-0.34815371122304039630535044125281274318695068359375;-0.2320934798606277826849009215948171913623809814453125;-0.8177263878639149385918472034973092377185821533203125;-0.4004659264562528964148668819689191877841949462890625;0.9852052407892359919827640624134801328182220458984375;-0.8790860570702019316513542435131967067718505859375;-0.7520229089538961186889309828984551131725311279296875;-0.486310433836135036500536443782038986682891845703125;0.0804089058620609531402578795677982270717620849609375;0.1939113091998303506358070080750621855258941650390625;-0.5694334409514791861539606543374247848987579345703125;0.041020374400621673061095862067304551601409912109375;-0.63187403134157360540257286629639565944671630859375;0.406940419921116625090462548541836440563201904296875;-0.638383341242963364692286631907336413860321044921875]
      mask Display: e = 0.06;c1 = [120 150 230]/255;c2 = ([120 150 230]+0)/383;c3 = ([120 150 230]+128)/383;patch([0 1 1 0],[0 0 1 1],c1);patch([0 1 1 1-e 1-e 0+e],[0 0 1 1-e 0+e 0+e],c2);patch([0 0 1 1-e 0+e 0+e],[0 1 1 1-e 1-e 0+e],c3);plot([0 1 1 0 0],[0 0 1 1 0]);disp('weights');
  "IW{3,2}(8,:)'" : Constant  Value=[0.065834360268933966864324247580952942371368408203125;-0.8587358519232417553013192446087487041950225830078125;-0.3757028777741744374196741773630492389202117919921875;0.387381441438808149513306489097885787487030029296875;-0.7623660854903249184388869252870790660381317138671875;0.578378113811186977955003385432064533233642578125;0.92802774539068533243835190660320222377777099609375;0.9315222419608926163192563763004727661609649658203125;-0.4453573868828100135175418472499586641788482666015625;-0.3239075921512151179371130638173781335353851318359375;-0.543094684532615445959891076199710369110107421875;0.265181424379623109643944189883768558502197265625;-0.8358578306212993691559631770360283553600311279296875;0.2872139959247246299156586246681399643421173095703125;0.0983004378392535738129254241357557475566864013671875]
      mask Display: e = 0.06;c1 = [120 150 230]/255;c2 = ([120 150 230]+0)/383;c3 = ([120 150 230]+128)/383;patch([0 1 1 0],[0 0 1 1],c1);patch([0 1 1 1-e 1-e 0+e],[0 0 1 1-e 0+e 0+e],c2);patch([0 0 1 1-e 0+e 0+e],[0 1 1 1-e 1-e 0+e],c3);plot([0 1 1 0 0],[0 0 1 1 0]);disp('weights');
  "IW{3,2}(9,:)'" : Constant  Value=[0.4281644156755806118752616384881548583507537841796875;-0.91161616821853908021466850186698138713836669921875;0.069575991587280672234783196472562849521636962890625;-0.6533917177043384594270492016221396625041961669921875;-0.919023562922785419715410171193070709705352783203125;-0.8818394943501479676939425189630128443241119384765625;0.244561023694448209653273806907236576080322265625;0.00809787728502708858968617278151214122772216796875;0.4934701959927141334816269591101445257663726806640625;0.1884537709115605697007822527666576206684112548828125;0.4950349159460785131159354932606220245361328125;-0.2472134903970317765242725727148354053497314453125;-0.026650106766705761174307554028928279876708984375;0.211677611937319820611946852295659482479095458984375;-0.474173165212278036051429808139801025390625]
      mask Display: e = 0.06;c1 = [120 150 230]/255;c2 = ([120 150 230]+0)/383;c3 = ([120 150 230]+128)/383;patch([0 1 1 0],[0 0 1 1],c1);patch([0 1 1 1-e 1-e 0+e],[0 0 1 1-e 0+e 0+e],c2);patch([0 0 1 1-e 0+e 0+e],[0 1 1 1-e 1-e 0+e],c3);plot([0 1 1 0 0],[0 0 1 1 0]);disp('weights');
  Mux : Mux  Inputs=15
      mask Display: e = 0.06;c1 = [120 150 230]/255;c2 = ([120 150 230]+0)/383;c3 = ([120 150 230]+128)/383;patch([0 1 1 0],[0 0 1 1],c1);patch([0 1 1 1-e 1-e 0+e],[0 0 1 1-e 0+e 0+e],c2);patch([0 0 1 1-e 0+e 0+e],[0 1 1 1-e 1-e 0+e],c3);plot([0 1 1 0 0],[0 0 1 1 0]);disp('Mux');
  dotprod{1..15} (15 alike) : neural/Weight Functions/dotprod
  "lz{3,2}" : Outport
      mask Display: e = 0.06;c1 = [120 230 180]/255;c2 = ([120 230 180]+0)/(256+128);c3 = ([120 230 180]+128)/(256+128);patch([0 1 1 0],[0 0 1 1],c1);patch([0 1 1 1-e 1-e 0+e],[0 0 1 1-e 0+e 0+e],c2);patch([0 0 1 1-e 0+e 0+e],[0 1 1 1-e 1-e 0+e],c3);plot([0 1 1 0 0],[0 0 1 1 0]);
  wires:
  "IW{3,2}(1,:)'"/1 -> dotprod1/1
  "ad{3,2}"/1 -> dotprod1/2, dotprod2/2, dotprod3/2, dotprod4/2, dotprod5/2, dotprod6/2, dotprod7/2, dotprod8/2, dotprod9/2, dotprod10/2, dotprod11/2, dotprod12/2, dotprod13/2, dotprod14/2, dotprod15/2
  dotprod1/1 -> Mux/1
  "IW{3,2}(2,:)'"/1 -> dotprod2/1
  dotprod2/1 -> Mux/2
  "IW{3,2}(3,:)'"/1 -> dotprod3/1
  dotprod3/1 -> Mux/3
  "IW{3,2}(4,:)'"/1 -> dotprod4/1
  dotprod4/1 -> Mux/4
  "IW{3,2}(5,:)'"/1 -> dotprod5/1
  dotprod5/1 -> Mux/5
  "IW{3,2}(6,:)'"/1 -> dotprod6/1
  dotprod6/1 -> Mux/6
  "IW{3,2}(7,:)'"/1 -> dotprod7/1
  dotprod7/1 -> Mux/7
  "IW{3,2}(8,:)'"/1 -> dotprod8/1
  dotprod8/1 -> Mux/8
  "IW{3,2}(9,:)'"/1 -> dotprod9/1
  dotprod9/1 -> Mux/9
  "IW{3,2}(10,:)'"/1 -> dotprod10/1
  dotprod10/1 -> Mux/10
  "IW{3,2}(11,:)'"/1 -> dotprod11/1
  dotprod11/1 -> Mux/11
  "IW{3,2}(12,:)'"/1 -> dotprod12/1
  dotprod12/1 -> Mux/12
  "IW{3,2}(13,:)'"/1 -> dotprod13/1
  dotprod13/1 -> Mux/13
  "IW{3,2}(14,:)'"/1 -> dotprod14/1
  dotprod14/1 -> Mux/14
  "IW{3,2}(15,:)'"/1 -> dotprod15/1
  dotprod15/1 -> Mux/15
  Mux/1 -> "lz{3,2}"/1

== system AFC_FFNN_trainbfg_15_15_15_15_ctr_Nor_July_15/Feed-Forward Neural Network/Layer 4/Delays 1 ==
  "p{4}" : Inport  PortDimensions=15
      mask Display: e = 0.06;c1 = [120 230 180]/255;c2 = ([120 230 180]+0)/(256+128);c3 = ([120 230 180]+128)/(256+128);patch([0 1 1 0],[0 0 1 1],c1);patch([0 1 1 1-e 1-e 0+e],[0 0 1 1-e 0+e 0+e],c2);patch([0 0 1 1-e 0+e 0+e],[0 1 1 1-e 1-e 0+e],c3);plot([0 1 1 0 0],[0 0 1 1 0]);
  mux : Mux  Inputs=1
      mask Display: e = 0.06;c1 = [120 150 230]/255;c2 = ([120 150 230]+0)/383;c3 = ([120 150 230]+128)/383;patch([0 1 1 0],[0 0 1 1],c1);patch([0 1 1 1-e 1-e 0+e],[0 0 1 1-e 0+e 0+e],c2);patch([0 0 1 1-e 0+e 0+e],[0 1 1 1-e 1-e 0+e],c3);plot([0 1 1 0 0],[0 0 1 1 0]);disp('Mux')
  "pd{4,3}" : Outport
      mask Display: e = 0.06;c1 = [120 230 180]/255;c2 = ([120 230 180]+0)/(256+128);c3 = ([120 230 180]+128)/(256+128);patch([0 1 1 0],[0 0 1 1],c1);patch([0 1 1 1-e 1-e 0+e],[0 0 1 1-e 0+e 0+e],c2);patch([0 0 1 1-e 0+e 0+e],[0 1 1 1-e 1-e 0+e],c3);plot([0 1 1 0 0],[0 0 1 1 0]);
  wires:
  "p{4}"/1 -> mux/1
  mux/1 -> "pd{4,3}"/1
